simulink model "ldo_demo"  (R2026a)
settings: Solver=ode4  StopTime=5e-05  FixedStep=1e-08
libraries: fl_lib x12, nesl_utility x6
settings Model: Creator=admin  LastModifiedBy=admin
settings DataIOCC: SaveFormat=StructureWithTime

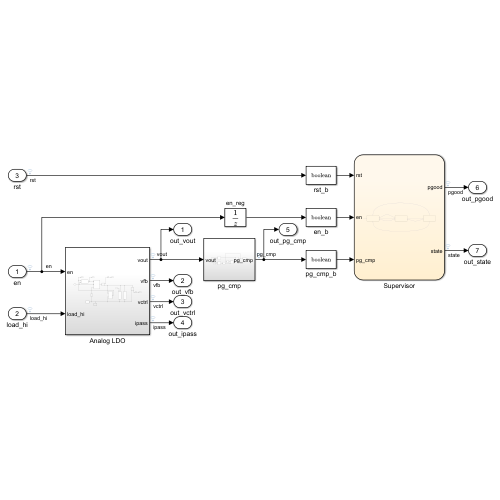
[thumbnail: Simulink's stored preview of the top-level diagram]
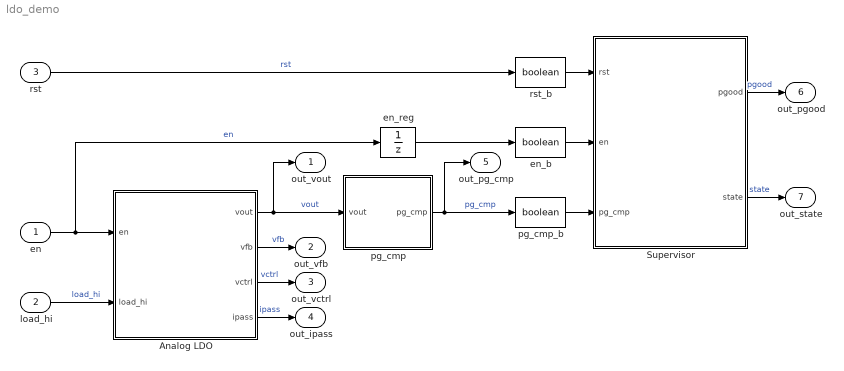
== system ldo_demo ==
  en : Inport  Interpolate=off
  load_hi : Inport  Port=2  Interpolate=off
  rst : Inport  Port=3  Interpolate=off
  Analog LDO : Subsystem
  Supervisor : Stateflow chart  TreatAsAtomicUnit=on
  en_b : DataTypeConversion  OutDataTypeStr=boolean  SaturateOnIntegerOverflow=off  RndMeth=Floor
  en_reg : UnitDelay  SampleTime=100e-9
  pg_cmp : Subsystem
  pg_cmp_b : DataTypeConversion  OutDataTypeStr=boolean  SaturateOnIntegerOverflow=off  RndMeth=Floor
  rst_b : DataTypeConversion  OutDataTypeStr=boolean  SaturateOnIntegerOverflow=off  RndMeth=Floor
  out_vout : Outport
  out_vfb : Outport  Port=2
  out_vctrl : Outport  Port=3
  out_ipass : Outport  Port=4
  out_pg_cmp : Outport  Port=5
  out_pgood : Outport  Port=6
  out_state : Outport  Port=7
  wires:
  Analog LDO/1(vout) -> out_vout/1, pg_cmp/1(vout)  "vout"
  Analog LDO/2(vfb) -> out_vfb/1  "vfb"
  Analog LDO/3(vctrl) -> out_vctrl/1  "vctrl"
  Analog LDO/4(ipass) -> out_ipass/1  "ipass"
  Supervisor/1(pgood) -> out_pgood/1  "pgood"
  Supervisor/2(state) -> out_state/1  "state"
  en/1 -> Analog LDO/1(en), en_reg/1  "en"
  en_b/1 -> Supervisor/2(en)
  load_hi/1 -> Analog LDO/2(load_hi)  "load_hi"
  pg_cmp/1(pg_cmp) -> out_pg_cmp/1, pg_cmp_b/1  "pg_cmp"
  pg_cmp_b/1 -> Supervisor/3(pg_cmp)
  rst/1 -> rst_b/1  "rst"
  rst_b/1 -> Supervisor/1(rst)
  en_reg/1 -> en_b/1

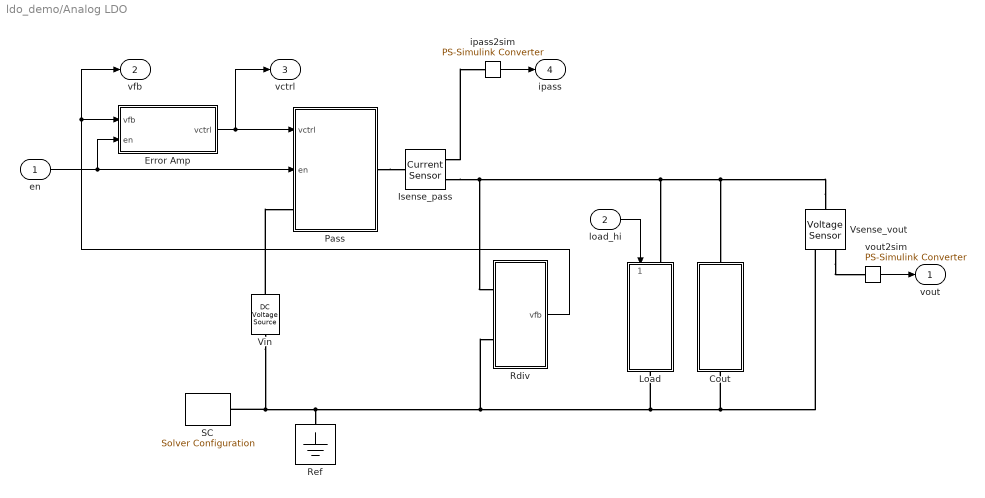
== system ldo_demo/Analog LDO ==
  en : Inport
  load_hi : Inport  Port=2
  Cout : Subsystem
  Error Amp : Subsystem
  Isense_pass : fl_lib/Electrical/Electrical Sensors/Current Sensor
  Load : Subsystem
  Pass : Subsystem
  Rdiv : Subsystem
  Ref : fl_lib/Electrical/Electrical Elements/Electrical Reference
  SC : nesl_utility/Solver Configuration  PhysicalDomain=network_engine_domain  SubClassName=solver  LeftPortType=input  RightPortType=generic  Tones=[]  Harmonics=[]  SimulateNoise=off  Profile=off  UseLocalSampling=off  EnableSwitchedLinearOptims=on  FrequencyDomain=off  UseCCode=off  RelTol=0.001  AbsTol=0.001  MinStep=1e-09  ToWorkspace=off  RevertToSquareIcSolve=off  NumHomotopyIterations=100  PhasorMode=off  PhasorModeNumHarmonics=1  ConsistencySolver=NEWTON_XTOL_AFTER_FTOL  CanonicalOrdering=CANONICAL  OptimizeIntermediates=OPTIMIZED  IndexReductionMethod=DerivativeReplacement  DoDC=off  ResidualTolerance=1e-09  ConsistencyTolSource=GLOBAL  ConsistencyAbsTol=0.001  ConsistencyRelTol=0.001  ConsistencyTolFactor=0.001  UseLocalSolver=off  LocalSolverChoice=NE_BACKWARD_EULER_ADVANCER  ResolveIndetEquations=on  FunctionEvalNumThread=1  LocalSolverSampleTime=0.001  DoFixedCost=off  MaxNonlinIter=3  MaxModeIter=2  ComputeImpulses=off  ImpulseIterations=2  LinearAlgebra=auto  LinearAlgebraNumThread=0  EquationFormulation=NE_TIME_EF  DelaysMemoryBudget=1024  AutomaticFiltering=on  FilteringTimeConstant=0.001  PartitionStorageMethod=AS_NEEDED  PartitionMemoryBudget=1024  PartitionMethod=ROBUST  MultibodyUseLocalSolver=off  MultibodyLocalSolverChoice=ODE1  MultibodyLocalSolverSampleTime=0.001
  Vin : fl_lib/Electrical/Electrical Sources/DC Voltage Source  v0=1.2 V
  Vsense_vout : fl_lib/Electrical/Electrical Sensors/Voltage Sensor
  ipass2sim : nesl_utility/PS-Simulink Converter  PhysicalDomain=network_engine_domain  SubClassName=ps_output  LeftPortType=input  RightPortType=output  PseudoPeriodic=off  Frequencies=[]  VectorFormat=inherit  Unit=A  AffineConversion=off
  vout2sim : nesl_utility/PS-Simulink Converter  PhysicalDomain=network_engine_domain  SubClassName=ps_output  LeftPortType=input  RightPortType=output  PseudoPeriodic=off  Frequencies=[]  VectorFormat=inherit  Unit=V  AffineConversion=off
  vout : Outport
  vfb : Outport  Port=2
  vctrl : Outport  Port=3
  ipass : Outport  Port=4
  wires:
  Error Amp/1(vctrl) -> vctrl/1, Pass/1(vctrl)
  Rdiv/1(vfb) -> vfb/1, Error Amp/1(vfb)
  en/1 -> Pass/2(en), Error Amp/2(en)
  ipass2sim/1 -> ipass/1
  load_hi/1 -> Load/1(load_hi)
  vout2sim/1 -> vout/1
  connections:
  Vsense_vout/RConn2 -- Vin/RConn1 -- SC/RConn1 -- Ref/LConn1 -- Rdiv/LConn2 -- Load/RConn1 -- Cout/RConn1
  Vsense_vout/LConn1 -- Isense_pass/RConn2 -- Rdiv/LConn1 -- Load/LConn1 -- Cout/LConn1
  Pass/RConn1 -- Isense_pass/LConn1
  Isense_pass/RConn1 -- ipass2sim/LConn1
  Vin/LConn1 -- Pass/LConn1
  Vsense_vout/RConn1 -- vout2sim/LConn1

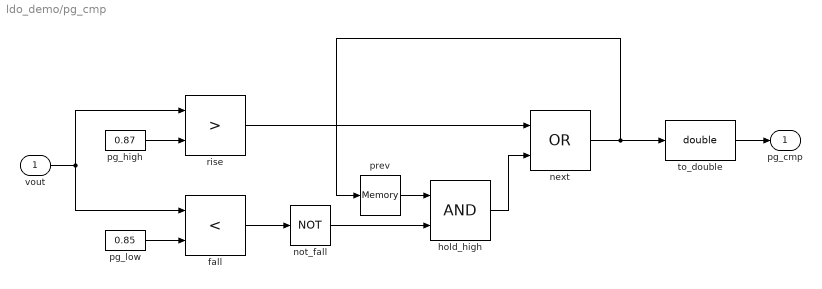
== system ldo_demo/pg_cmp ==
  vout : Inport
  fall : RelationalOperator  Operator=<  OutDataTypeStr=boolean  RndMeth=Simplest  InputSameDT=off
  hold_high : Logic  AllPortsSameDT=off  OutDataTypeStr=boolean
  next : Logic  Operator=OR  AllPortsSameDT=off  OutDataTypeStr=boolean
  not_fall : Logic  Operator=NOT  AllPortsSameDT=off  OutDataTypeStr=boolean
  pg_high : Constant  Value=0.87
  pg_low : Constant  Value=0.85
  prev : Memory
  rise : RelationalOperator  Operator=>  OutDataTypeStr=boolean  RndMeth=Simplest  InputSameDT=off
  to_double : DataTypeConversion  OutDataTypeStr=double  SaturateOnIntegerOverflow=off  RndMeth=Floor
  pg_cmp : Outport
  wires:
  fall/1 -> not_fall/1
  hold_high/1 -> next/2
  next/1 -> prev/1, to_double/1
  not_fall/1 -> hold_high/2
  pg_high/1 -> rise/2
  pg_low/1 -> fall/2
  prev/1 -> hold_high/1
  rise/1 -> next/1
  to_double/1 -> pg_cmp/1
  vout/1 -> rise/1, fall/1

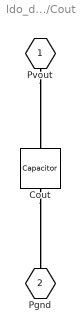
== system ldo_demo/Analog LDO/Cout ==
  Cout : fl_lib/Electrical/Electrical Elements/Capacitor  c=10 nF  r=1e-6 Ohm  g=0 1/Ohm  i_specify=off  i_priority=None  i=0 A  i_nominal_specify=off  i_nominal_value=1  i_nominal_unit=A  v_specify=off  v_priority=None  v=0 V  v_nominal_specify=off  v_nominal_value=1  v_nominal_unit=V  vc_specify=off  vc_priority=High  vc=0 V  vc_nominal_specify=off  vc_nominal_value=1  vc_nominal_unit=V
  Pvout : PMIOPort  Side=Left
  Pgnd : PMIOPort  Port=2  Side=Right
  connections:
  Pvout/RConn1 -- Cout/LConn1
  Cout/RConn1 -- Pgnd/RConn1

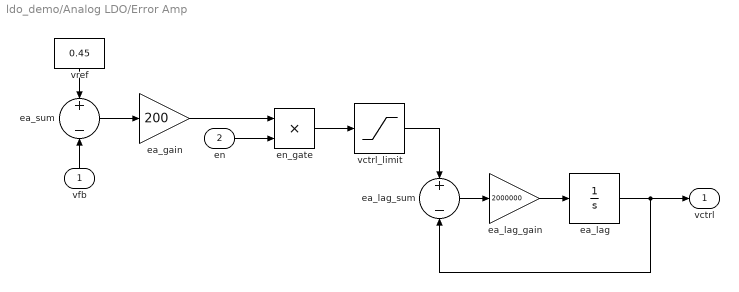
== system ldo_demo/Analog LDO/Error Amp ==
  vfb : Inport
  en : Inport  Port=2
  ea_gain : Gain  Gain=200
  ea_lag : Integrator
  ea_lag_gain : Gain  Gain=2000000
  ea_lag_sum : Sum  Inputs=+-
  ea_sum : Sum  Inputs=+-
  en_gate : Product  Inputs=**
  vctrl_limit : Saturate  UpperLimit=1  LowerLimit=0
  vref : Constant  Value=0.45
  vctrl : Outport
  wires:
  ea_gain/1 -> en_gate/1
  ea_lag/1 -> ea_lag_sum/2, vctrl/1
  ea_lag_gain/1 -> ea_lag/1
  ea_lag_sum/1 -> ea_lag_gain/1
  ea_sum/1 -> ea_gain/1
  en/1 -> en_gate/2
  en_gate/1 -> vctrl_limit/1
  vctrl_limit/1 -> ea_lag_sum/1
  vfb/1 -> ea_sum/2
  vref/1 -> ea_sum/1

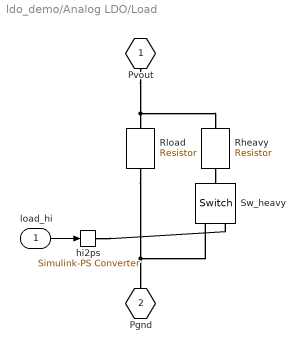
== system ldo_demo/Analog LDO/Load ==
  load_hi : Inport
  Rheavy : fl_lib/Electrical/Electrical Elements/Resistor  R=360 Ohm  i_specify=off  i_priority=None  i=0 A  i_nominal_specify=off  i_nominal_value=1  i_nominal_unit=A  v_specify=off  v_priority=None  v=0 V  v_nominal_specify=off  v_nominal_value=1  v_nominal_unit=V
  Rload : fl_lib/Electrical/Electrical Elements/Resistor  R=1800 Ohm  i_specify=off  i_priority=None  i=0 A  i_nominal_specify=off  i_nominal_value=1  i_nominal_unit=A  v_specify=off  v_priority=None  v=0 V  v_nominal_specify=off  v_nominal_value=1  v_nominal_unit=V
  Sw_heavy : fl_lib/Electrical/Electrical Elements/Switch  R_closed=1e-06 Ohm  G_open=1e-12 1/Ohm  Threshold=0.5  i_specify=off  i_priority=None  i=0 A  i_nominal_specify=off  i_nominal_value=1  i_nominal_unit=A  v_specify=off  v_priority=None  v=0 V  v_nominal_specify=off  v_nominal_value=1  v_nominal_unit=V
  hi2ps : nesl_utility/Simulink-PS Converter  PhysicalDomain=network_engine_domain  SubClassName=ps_input  LeftPortType=input  RightPortType=output  PseudoPeriodic=off  Frequencies=[]  NoiseDistribution=none  NoiseParameters=[]  Unit=1  AffineConversion=off  FilteringAndDerivatives=provide  SimscapeFilterOrder=1  InputFilterTimeConstant=0.001  UdotUserProvided=0
  Pvout : PMIOPort  Side=Left
  Pgnd : PMIOPort  Port=2  Side=Right
  wires:
  load_hi/1 -> hi2ps/1
  connections:
  Sw_heavy/RConn2 -- Rload/RConn1 -- Pgnd/RConn1
  Rheavy/LConn1 -- Pvout/RConn1 -- Rload/LConn1
  Rheavy/RConn1 -- Sw_heavy/LConn1
  hi2ps/RConn1 -- Sw_heavy/RConn1

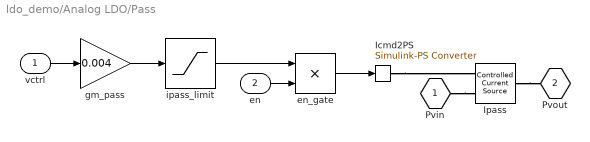
== system ldo_demo/Analog LDO/Pass ==
  vctrl : Inport
  en : Inport  Port=2
  Icmd2PS : nesl_utility/Simulink-PS Converter  PhysicalDomain=network_engine_domain  SubClassName=ps_input  LeftPortType=input  RightPortType=output  PseudoPeriodic=off  Frequencies=[]  NoiseDistribution=none  NoiseParameters=[]  Unit=A  AffineConversion=off  FilteringAndDerivatives=provide  SimscapeFilterOrder=1  InputFilterTimeConstant=0.001  UdotUserProvided=0
  Ipass : fl_lib/Electrical/Electrical Sources/Controlled Current Source
  en_gate : Product  Inputs=**
  gm_pass : Gain  Gain=0.004
  ipass_limit : Saturate  UpperLimit=0.005  LowerLimit=0
  Pvin : PMIOPort  Side=Left
  Pvout : PMIOPort  Port=2  Side=Right
  wires:
  en/1 -> en_gate/2
  en_gate/1 -> Icmd2PS/1
  gm_pass/1 -> ipass_limit/1
  ipass_limit/1 -> en_gate/1
  vctrl/1 -> gm_pass/1
  connections:
  Icmd2PS/RConn1 -- Ipass/RConn1
  Ipass/LConn1 -- Pvout/RConn1
  Pvin/RConn1 -- Ipass/RConn2

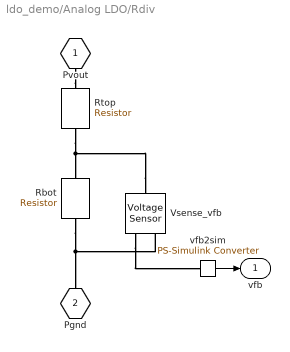
== system ldo_demo/Analog LDO/Rdiv ==
  Rbot : fl_lib/Electrical/Electrical Elements/Resistor  R=100000 Ohm  i_specify=off  i_priority=None  i=0 A  i_nominal_specify=off  i_nominal_value=1  i_nominal_unit=A  v_specify=off  v_priority=None  v=0 V  v_nominal_specify=off  v_nominal_value=1  v_nominal_unit=V
  Rtop : fl_lib/Electrical/Electrical Elements/Resistor  R=100000 Ohm  i_specify=off  i_priority=None  i=0 A  i_nominal_specify=off  i_nominal_value=1  i_nominal_unit=A  v_specify=off  v_priority=None  v=0 V  v_nominal_specify=off  v_nominal_value=1  v_nominal_unit=V
  Vsense_vfb : fl_lib/Electrical/Electrical Sensors/Voltage Sensor
  vfb2sim : nesl_utility/PS-Simulink Converter  PhysicalDomain=network_engine_domain  SubClassName=ps_output  LeftPortType=input  RightPortType=output  PseudoPeriodic=off  Frequencies=[]  VectorFormat=inherit  Unit=V  AffineConversion=off
  Pvout : PMIOPort  Side=Left
  Pgnd : PMIOPort  Port=2  Side=Left
  vfb : Outport
  wires:
  vfb2sim/1 -> vfb/1
  connections:
  Vsense_vfb/RConn2 -- Rbot/RConn1 -- Pgnd/RConn1
  Pvout/RConn1 -- Rtop/LConn1
  Vsense_vfb/LConn1 -- Rtop/RConn1 -- Rbot/LConn1
  Vsense_vfb/RConn1 -- vfb2sim/LConn1

== stateflow chart ldo_demo/Supervisor ==
  settings: updateMethod=DISCRETE  sampleTime=1e-07  executeAtInitialization=1
  state OFF
    en: pgood = 0; state = 0;
  state WAIT
    en: pgood = 0; state = 1;
  state ON
    en: pgood = 1; state = 2;
  ON -> OFF [order 1] : [rst]
  WAIT -> OFF [order 1] : [rst]
  OFF -> WAIT : [en && ~rst]
  WAIT -> ON [order 3] : [duration(pg_cmp, sec) >= 1.95e-06]
  (default) -> OFF
  WAIT -> OFF [order 2] : [~en]
  ON -> WAIT [order 3] : [~pg_cmp]
  ON -> OFF [order 2] : [~en]
  data: rst input boolean; en input boolean; pg_cmp input boolean; pgood output double; state output double
